simulink model "uacs_lqr"  (R2024a)
settings: Solver=ode4  StartTime=0.0  StopTime=sim_t_end  FixedStep=sim_ts_ctrl  RelTol=1e-3
undefined symbols (not defined in the file): DiscIntNeverNeededParam, sim_c_zero, sim_G_surf, sim_lqr_C_lat, sim_lqr_C_long, sim_lqr_K_lat, sim_lqr_K_long, sim_lqr_Tref_lat, sim_lqr_Tref_long, sim_lqr_Uff_lat, sim_lqr_Uff_long, sim_lqr_xop_lat, sim_lqr_xop_long, sim_lqr_zlim_lat, sim_lqr_zlim_lat_neg, sim_lqr_zlim_long, sim_lqr_zlim_long_neg, sim_T_trim, sim_ts_ctrl, sim_u_trim_surf
settings Model: Creator=Ash Trailer  LastModifiedBy=Ash Trailer
settings DataIOCC: SaveFormat=StructureWithTime
settings DebuggingCC: AlgebraicLoopMsg=error

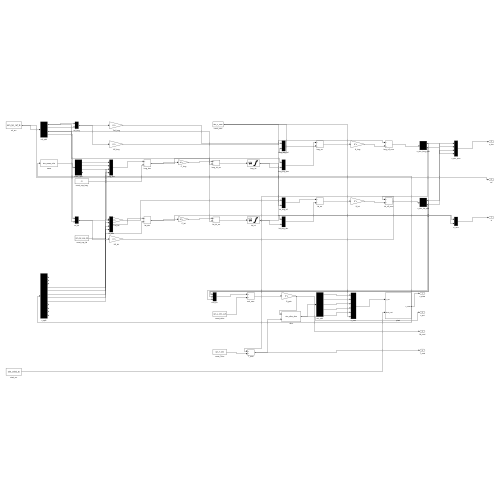
[thumbnail: Simulink's stored preview of the top-level diagram]
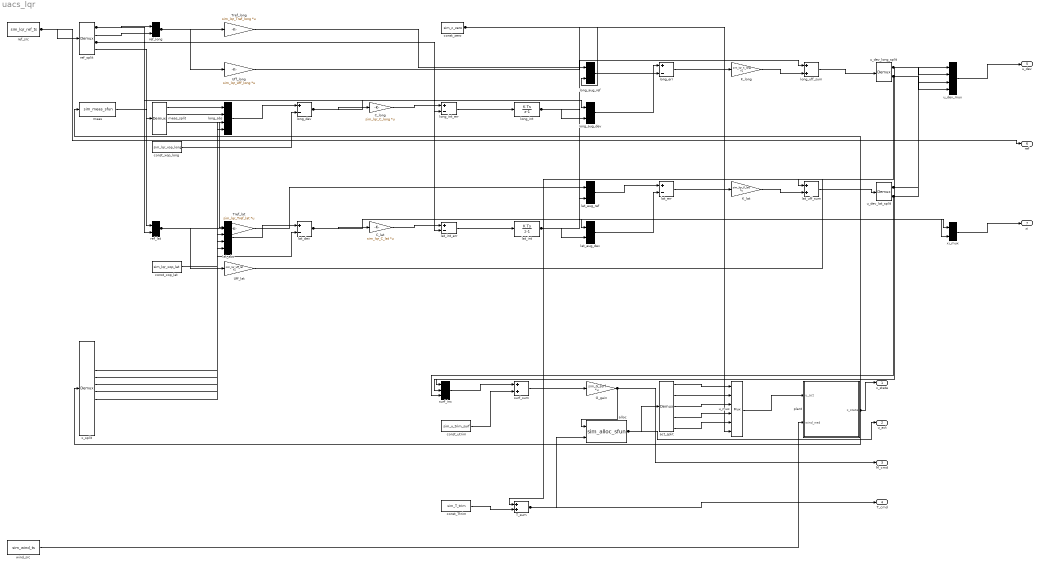
== system uacs_lqr ==
  C_lat : Gain  Gain=sim_lqr_C_lat  Multiplication=Matrix(K*u)
  C_long : Gain  Gain=sim_lqr_C_long  Multiplication=Matrix(K*u)
  G_gain : Gain  Gain=sim_G_surf  Multiplication=Matrix(K*u)
  K_lat : Gain  Gain=sim_lqr_K_lat  Multiplication=Matrix(K*u)
  K_long : Gain  Gain=sim_lqr_K_long  Multiplication=Matrix(K*u)
  T_sum : Sum
  Tref_lat : Gain  Gain=sim_lqr_Tref_lat  Multiplication=Matrix(K*u)
  Tref_long : Gain  Gain=sim_lqr_Tref_long  Multiplication=Matrix(K*u)
  Uff_lat : Gain  Gain=sim_lqr_Uff_lat  Multiplication=Matrix(K*u)
  Uff_long : Gain  Gain=sim_lqr_Uff_long  Multiplication=Matrix(K*u)
  act_split : Demux  Outputs=5
  alloc : M-S-Function  FunctionName=sim_alloc_sfun
  const_Ttrim : Constant  Value=sim_T_trim
  const_utrim : Constant  Value=sim_u_trim_surf
  const_xop_lat : Constant  Value=sim_lqr_xop_lat
  const_xop_long : Constant  Value=sim_lqr_xop_long
  const_zero : Constant  Value=sim_c_zero
  lat_abs : Mux
  lat_aug_dev : Mux  Inputs=2
  lat_aug_ref : Mux  Inputs=2
  lat_dev : Sum  Inputs=+-
  lat_err : Sum  Inputs=+-
  lat_int : DiscreteIntegrator  gainval=sim_c_one  SampleTime=sim_ts_ctrl  LimitOutput=on  UpperSaturationLimit=sim_lqr_zlim_lat  LowerSaturationLimit=sim_lqr_zlim_lat_neg  ICPrevOutput=DiscIntNeverNeededParam  ICPrevScaledInput=DiscIntNeverNeededParam
  lat_int_err : Sum  Inputs=+-
  lat_uff_sum : Sum
  long_abs : Mux
  long_aug_dev : Mux  Inputs=2
  long_aug_ref : Mux  Inputs=2
  long_dev : Sum  Inputs=+-
  long_err : Sum  Inputs=+-
  long_int : DiscreteIntegrator  gainval=sim_c_one  SampleTime=sim_ts_ctrl  LimitOutput=on  UpperSaturationLimit=sim_lqr_zlim_long  LowerSaturationLimit=sim_lqr_zlim_long_neg  ICPrevOutput=DiscIntNeverNeededParam  ICPrevScaledInput=DiscIntNeverNeededParam
  long_int_err : Sum  Inputs=+-
  long_uff_sum : Sum
  meas : M-S-Function  FunctionName=sim_meas_sfun
  meas_split : Demux
  plant : Subsystem
  ref_lat : Mux  Inputs=2
  ref_long : Mux  Inputs=2
  ref_split : Demux
  ref_src : FromWorkspace  VariableName=sim_lqr_ref_ts  OutputAfterFinalValue=Holding final value
  surf_inc : Mux  Inputs=3
  surf_sum : Sum
  u_dev_lat_split : Demux  Outputs=2
  u_dev_long_split : Demux  Outputs=2
  u_dev_mux : Mux
  u_mux : Mux  Inputs=6
  wind_src : FromWorkspace  VariableName=sim_wind_ts  OutputAfterFinalValue=Holding final value
  x_split : Demux  Outputs=12
  xi_mux : Mux  Inputs=2
  x_state : Outport
  u_act : Outport  Port=2
  M_cmd : Outport  Port=3
  T_cmd : Outport  Port=4
  u_dev : Outport  Port=5
  ref : Outport  Port=6
  xi : Outport  Port=7
  wires:
  ref_src/1 -> ref_split/1, ref/1
  ref_split/1 -> ref_long/1, long_int_err/2
  ref_split/2 -> ref_long/2
  ref_long/1 -> Tref_long/1, Uff_long/1
  ref_split/4 -> ref_lat/1
  ref_split/3 -> ref_lat/2, lat_int_err/2
  ref_lat/1 -> Tref_lat/1, Uff_lat/1
  meas/1 -> meas_split/1
  meas_split/1 -> long_abs/1
  meas_split/2 -> long_abs/2
  meas_split/3 -> lat_abs/1
  x_split/5 -> long_abs/3
  x_split/8 -> long_abs/4
  x_split/4 -> lat_abs/2
  x_split/6 -> lat_abs/3
  x_split/7 -> lat_abs/4
  long_abs/1 -> long_dev/1
  const_xop_long/1 -> long_dev/2
  long_dev/1 -> C_long/1, long_aug_dev/1
  C_long/1 -> long_int_err/1
  long_int_err/1 -> long_int/1
  long_int/1 -> long_aug_dev/2, xi_mux/1
  Tref_long/1 -> long_aug_ref/1
  const_zero/1 -> long_aug_ref/2, lat_aug_ref/2, u_mux/6
  long_aug_ref/1 -> long_err/1
  long_aug_dev/1 -> long_err/2
  long_err/1 -> K_long/1
  K_long/1 -> long_uff_sum/2
  Uff_long/1 -> long_uff_sum/1
  long_uff_sum/1 -> u_dev_long_split/1
  lat_abs/1 -> lat_dev/1
  const_xop_lat/1 -> lat_dev/2
  lat_dev/1 -> C_lat/1, lat_aug_dev/1
  C_lat/1 -> lat_int_err/1
  lat_int_err/1 -> lat_int/1
  lat_int/1 -> lat_aug_dev/2, xi_mux/2
  Tref_lat/1 -> lat_aug_ref/1
  lat_aug_ref/1 -> lat_err/1
  lat_aug_dev/1 -> lat_err/2
  lat_err/1 -> K_lat/1
  K_lat/1 -> lat_uff_sum/2
  Uff_lat/1 -> lat_uff_sum/1
  lat_uff_sum/1 -> u_dev_lat_split/1
  u_dev_lat_split/1 -> surf_inc/1, u_dev_mux/1
  u_dev_long_split/1 -> surf_inc/2, u_dev_mux/2
  u_dev_lat_split/2 -> surf_inc/3, u_dev_mux/3
  surf_inc/1 -> surf_sum/1
  const_utrim/1 -> surf_sum/2
  surf_sum/1 -> G_gain/1
  G_gain/1 -> alloc/1, M_cmd/1
  u_dev_long_split/2 -> T_sum/1, u_dev_mux/4
  const_Ttrim/1 -> T_sum/2
  T_sum/1 -> alloc/2, T_cmd/1
  alloc/1 -> act_split/1, u_act/1
  act_split/1 -> u_mux/1
  act_split/2 -> u_mux/2
  act_split/3 -> u_mux/3
  act_split/4 -> u_mux/4
  act_split/5 -> u_mux/5
  u_mux/1 -> plant/1(u_act)
  wind_src/1 -> plant/2(wind_ned)
  plant/1(x_state) -> x_state/1, x_split/1, meas/1
  u_dev_mux/1 -> u_dev/1
  xi_mux/1 -> xi/1

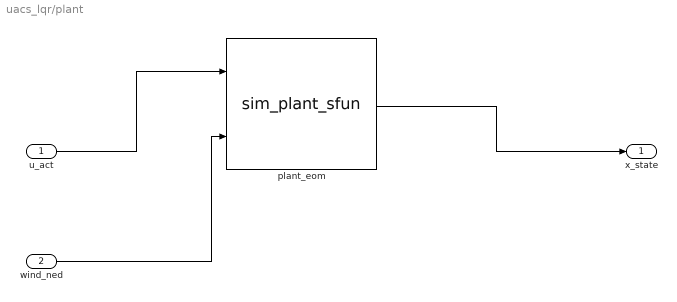
== system uacs_lqr/plant ==
  u_act : Inport
  wind_ned : Inport  Port=2
  plant_eom : M-S-Function  FunctionName=sim_plant_sfun
  x_state : Outport
  wires:
  u_act/1 -> plant_eom/1
  wind_ned/1 -> plant_eom/2
  plant_eom/1 -> x_state/1
